simulink model "TestCinematicoZ"  (R2022b)
settings: Solver=FixedStepDiscrete  StartTime=0.0  StopTime=inf  FixedStep=0.01  RelTol=1e-3  EnableMultiTasking=on
model workspace (MAT data in the model file):
  d = 0.15
settings Model: ExtModeTrigDuration=2  Creator=miriamfreiriasanjuan  LastModifiedBy=miriamfreiriasanjuan
settings OptimizationCC: EnhancedBackFolding=on  PassReuseOutputArgsAs=Individual arguments  ZeroExternalMemoryAtStartup=off  ZeroInternalMemoryAtStartup=off  MaxStackSize=64  OptimizeBlockOrder=speed  DifferentSizesBufferReuse=on  EfficientTunableParamExpr=on
settings DebuggingCC: ParameterTunabilityLossMsg=error
settings HardwareCC: ProdBitPerInt=16  ProdBitPerPointer=16  ProdBitPerSizeT=16  ProdBitPerPtrDiffT=16  ProdLargestAtomicFloat=None  ProdWordSize=8  ProdHWDeviceType=Atmel->AVR
settings SFSimCC: MATLABDynamicMemAlloc=off
settings RTWCC: Description=Embedded Coder  SystemTargetFile=ert.tlc  HardwareBoard=Arduino Mega 2560  TLCOptions=-aInlineSetEventsForThisBaseRateFcn=TLC_FALSE -aSuppressMultiTaskScheduler=TLC_FALSE -aRateBasedStepFcn=1  TemplateMakefile=ert_default_tmf  Toolchain=Arduino AVR  BuildConfiguration=Faster Runs
settings CodeAppCC: ForceParamTrailComments=on  IgnoreCustomStorageClasses=off  OperatorAnnotations=on  SimulinkDataObjDesc=on  SFDataObjDesc=on  InsertBlockDesc=on
settings ERTTargetCC: SupportContinuousTime=on  SupportVariableSizeSignals=on  ExtModeTransport=3  ExtModeStaticAlloc=on  ExtModeAutomaticAllocSize=off  ExtModeStaticAllocSize=2048  ExtModeMexFile=ext_xcp  ExtModeIntrfLevel=Level2 - Open

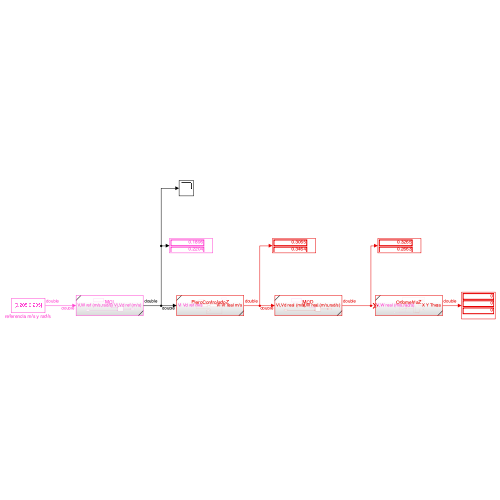
[thumbnail: Simulink's stored preview of the top-level diagram]
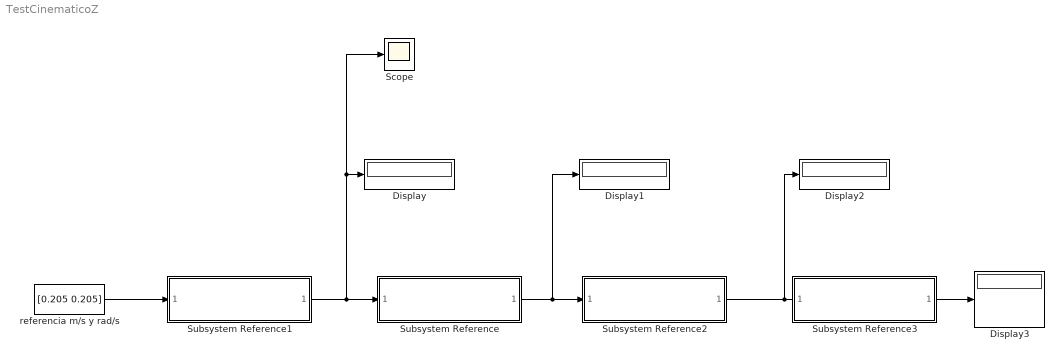
== system TestCinematicoZ ==
  Display{,1..3} (4 alike) : Display
  Scope : Scope
  Subsystem Reference : Subsystem  ReferencedSubsystem=PieroControladoZ
  Subsystem Reference1 : Subsystem  ReferencedSubsystem=MCI
  Subsystem Reference2 : Subsystem  ReferencedSubsystem=MCD
  Subsystem Reference3 : Subsystem  ReferencedSubsystem=OdometriaZ
  referencia m/s y rad/s : Constant  Value=[0.205 0.205]
  wires:
  Subsystem Reference2/1 -> Display2/1
  referencia m/s y rad/s/1 -> Subsystem Reference1/1
  Subsystem Reference3/1 -> Display3/1
  Subsystem Reference/1 -> Display1/1, Subsystem Reference2/1
  Subsystem Reference1/1 -> Subsystem Reference/1, Scope/1, Display/1
